simulink model "PassingDeadzone"  (R2023b)
settings: Solver=VariableStepAuto  StartTime=0.0  StopTime=20.0  FixedStep=.1  MaxStep=0.1  RelTol=1e-3
undefined symbols (not defined in the file or in its folder): Blue_Hub_LeftX, Blue_Hub_LeftY, Blue_Hub_RightX, Blue_Hub_RightY, Field_Length, Field_Length_Half, Field_Width, Rebuilt_Des_Gyro_Shoot_Offset
libraries: simulink_extras x3
settings Model: Creator=FIRSTMentor  LastModifiedBy=FIRSTMentor

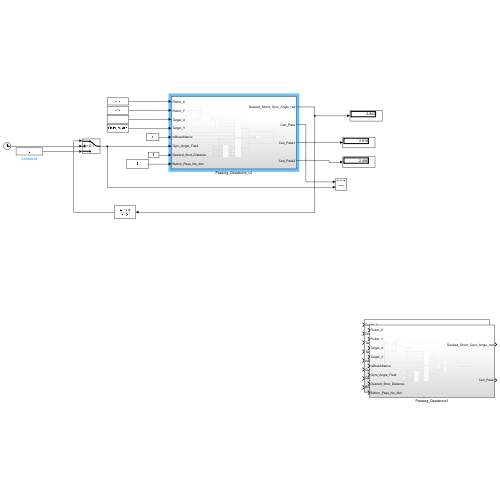
[thumbnail: Simulink's stored preview of the top-level diagram]
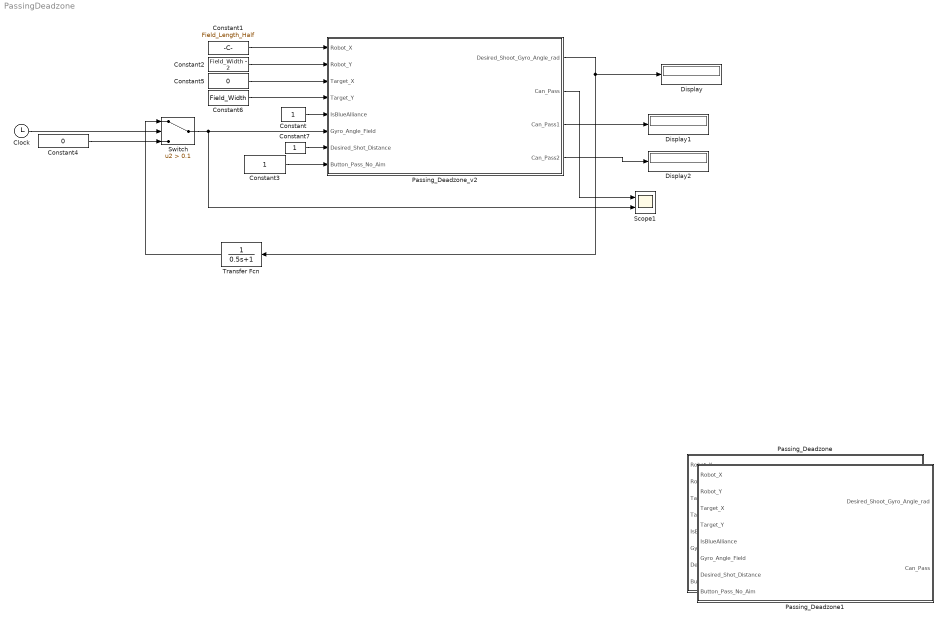
== system PassingDeadzone ==
  Clock : Clock
  Constant : Constant
  Constant1 : Constant  Value=Field_Length_Half
  Constant2 : Constant  Value=Field_Width - 2
  Constant3 : Constant
  Constant4 : Constant  Value=0
  Constant5 : Constant  Value=0
  Constant6 : Constant  Value=Field_Width
  Constant7 : Constant
  Display : Display
  Display1 : Display
  Display2 : Display
  Passing_Deadzone : Subsystem
  Passing_Deadzone1 : Subsystem
  Passing_Deadzone_v2 : Subsystem
  Scope1 : Scope  NumInputPorts=2
  Switch : Switch  Criteria=u2 > Threshold  Threshold=0.1  SaturateOnIntegerOverflow=off  InputSameDT=off
  Transfer Fcn : TransferFcn  Denominator=[0.5 1]
  wires:
  Constant/1 -> Passing_Deadzone_v2/5(IsBlueAlliance)
  Passing_Deadzone_v2/1(Desired_Shoot_Gyro_Angle_rad) -> Transfer Fcn/1, Display/1
  Passing_Deadzone_v2/2(Can_Pass) -> Scope1/1
  Constant3/1 -> Passing_Deadzone_v2/8(Button_Pass_No_Aim)
  Clock/1 -> Switch/2
  Constant4/1 -> Switch/3
  Transfer Fcn/1 -> Switch/1
  Switch/1 -> Scope1/2, Passing_Deadzone_v2/6(Gyro_Angle_Field)
  Constant1/1 -> Passing_Deadzone_v2/1(Robot_X)
  Constant2/1 -> Passing_Deadzone_v2/2(Robot_Y)
  Constant5/1 -> Passing_Deadzone_v2/3(Target_X)
  Constant6/1 -> Passing_Deadzone_v2/4(Target_Y)
  Constant7/1 -> Passing_Deadzone_v2/7(Desired_Shot_Distance)
  Passing_Deadzone_v2/3(Can_Pass1) -> Display1/1
  Passing_Deadzone_v2/4(Can_Pass2) -> Display2/1

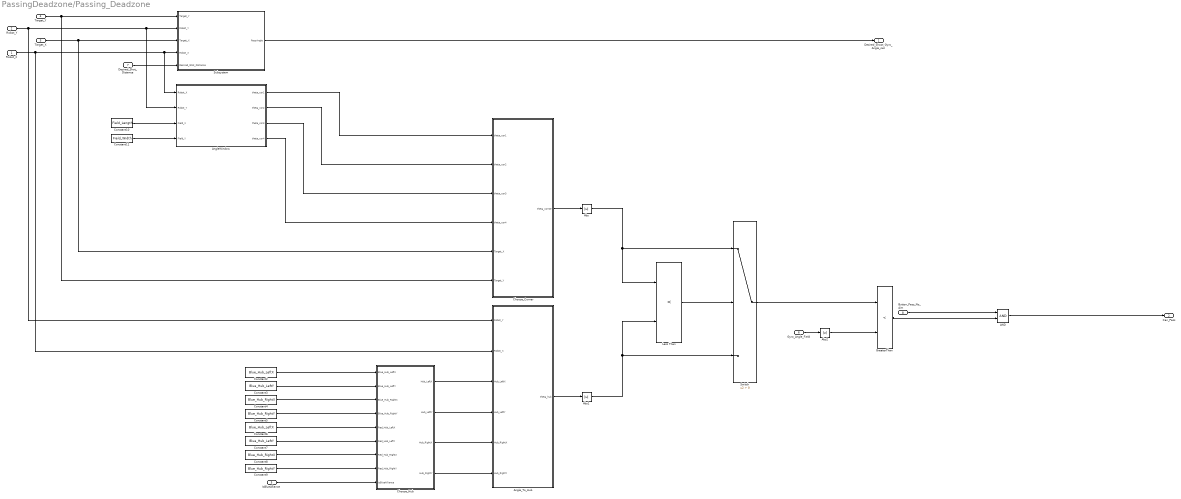
== system PassingDeadzone/Passing_Deadzone ==
  Robot_X : Inport
  Robot_Y : Inport  Port=2
  Target_X : Inport  Port=3
  Target_Y : Inport  Port=4
  IsBlueAlliance : Inport  Port=5
  Gyro_Angle_Field : Inport  Port=6
  Desired_Shot_Distance : Inport  Port=7
  Button_Pass_No_Aim : Inport  Port=8
  AND : Logic  AllPortsSameDT=off  OutDataTypeStr=boolean
  Abs : Abs  SaturateOnIntegerOverflow=off
  Abs1 : Abs  SaturateOnIntegerOverflow=off
  Abs2 : Abs  SaturateOnIntegerOverflow=off
  AngleWindow : Subsystem
  Angle_To_Hub : Subsystem
  Choose_Corner : Subsystem
  Choose_Hub : Subsystem
  Constant10 : Constant  Value=Field_Length
  Constant11 : Constant  Value=Field_Width
  Constant2 : Constant  Value=Blue_Hub_LeftX
  Constant3 : Constant  Value=Blue_Hub_LeftY
  Constant4 : Constant  Value=Blue_Hub_RightX
  Constant5 : Constant  Value=Blue_Hub_RightY
  Constant6 : Constant  Value=Blue_Hub_LeftX
  Constant7 : Constant  Value=Blue_Hub_LeftY
  Constant8 : Constant  Value=Blue_Hub_RightX
  Constant9 : Constant  Value=Blue_Hub_RightY
  GreaterThan : RelationalOperator  Operator=<  OutDataTypeStr=boolean  RndMeth=Simplest  InputSameDT=off
  Less Than : RelationalOperator  Operator=<  OutDataTypeStr=boolean  RndMeth=Simplest  InputSameDT=off
  Subsystem : Subsystem
  Switch : Switch  Criteria=u2 > Threshold  SaturateOnIntegerOverflow=off  InputSameDT=off
  Desired_Shoot_Gyro_Angle_rad : Outport
  Can_Pass : Outport  Port=2
  wires:
  Target_Y/1 -> Choose_Corner/6(Target_Y), Subsystem/1(Target_Y)
  Robot_Y/1 -> Angle_To_Hub/1(Robot_Y), AngleWindow/2(Robot_Y), Subsystem/2(Robot_Y)
  Target_X/1 -> Choose_Corner/5(Target_X), Subsystem/3(Target_X)
  Robot_X/1 -> AngleWindow/1(Robot_X), Subsystem/4(Robot_X), Angle_To_Hub/2(Robot_X)
  Constant10/1 -> AngleWindow/3(Field_X)
  AngleWindow/1(theta_cor1) -> Choose_Corner/1(theta_cor1)
  AngleWindow/2(theta_cor2) -> Choose_Corner/2(theta_cor2)
  AngleWindow/3(theta_cor3) -> Choose_Corner/3(theta_cor3)
  AngleWindow/4(theta_cor4) -> Choose_Corner/4(theta_cor4)
  Constant2/1 -> Choose_Hub/1(Blue_Hub_LeftX)
  Constant4/1 -> Choose_Hub/3(Blue_Hub_RightX)
  Constant5/1 -> Choose_Hub/4(Blue_Hub_RightY)
  Constant6/1 -> Choose_Hub/5(Red_Hub_LeftX)
  Constant7/1 -> Choose_Hub/6(Red_Hub_LeftY)
  Constant8/1 -> Choose_Hub/7(Red_Hub_RightX)
  Constant9/1 -> Choose_Hub/8(Red_Hub_RightY)
  IsBlueAlliance/1 -> Choose_Hub/9(IsBlueAlliance)
  Choose_Hub/1(Hub_LeftX) -> Angle_To_Hub/3(Hub_LeftX)
  Choose_Hub/2(Hub_LeftY) -> Angle_To_Hub/4(Hub_LeftY)
  Choose_Hub/3(Hub_RightX) -> Angle_To_Hub/5(Hub_RightX)
  Choose_Hub/4(Hub_RightY) -> Angle_To_Hub/6(Hub_RightY)
  Choose_Corner/1(theta_corner) -> Abs/1
  Angle_To_Hub/1(theta_hub) -> Abs1/1
  Abs/1 -> Switch/1, Less Than/1
  Abs1/1 -> Switch/3, Less Than/2
  Less Than/1 -> Switch/2
  Switch/1 -> GreaterThan/1
  Gyro_Angle_Field/1 -> Abs2/1
  Subsystem/1(PassAngle) -> Desired_Shoot_Gyro_Angle_rad/1
  Abs2/1 -> GreaterThan/2
  Constant3/1 -> Choose_Hub/2(Blue_Hub_LeftY)
  Constant11/1 -> AngleWindow/4(Field_Y)
  Desired_Shot_Distance/1 -> Subsystem/5(Desired_Shot_Distance)
  AND/1 -> Can_Pass/1
  Button_Pass_No_Aim/1 -> AND/1
  GreaterThan/1 -> AND/2

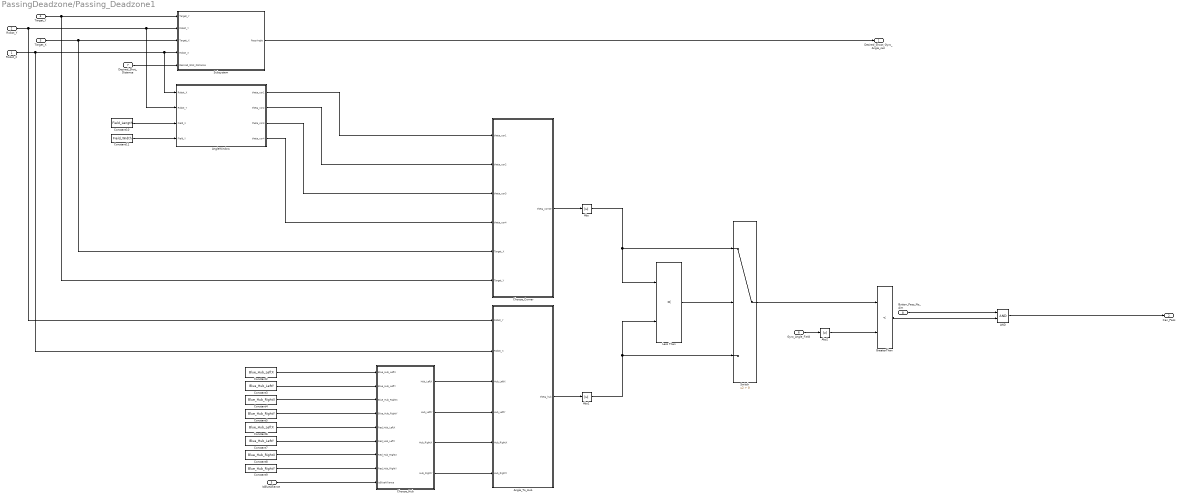
== system PassingDeadzone/Passing_Deadzone1 ==
  Robot_X : Inport
  Robot_Y : Inport  Port=2
  Target_X : Inport  Port=3
  Target_Y : Inport  Port=4
  IsBlueAlliance : Inport  Port=5
  Gyro_Angle_Field : Inport  Port=6
  Desired_Shot_Distance : Inport  Port=7
  Button_Pass_No_Aim : Inport  Port=8
  AND : Logic  AllPortsSameDT=off  OutDataTypeStr=boolean
  Abs : Abs  SaturateOnIntegerOverflow=off
  Abs1 : Abs  SaturateOnIntegerOverflow=off
  Abs2 : Abs  SaturateOnIntegerOverflow=off
  AngleWindow : Subsystem
  Angle_To_Hub : Subsystem
  Choose_Corner : Subsystem
  Choose_Hub : Subsystem
  Constant10 : Constant  Value=Field_Length
  Constant11 : Constant  Value=Field_Width
  Constant2 : Constant  Value=Blue_Hub_LeftX
  Constant3 : Constant  Value=Blue_Hub_LeftY
  Constant4 : Constant  Value=Blue_Hub_RightX
  Constant5 : Constant  Value=Blue_Hub_RightY
  Constant6 : Constant  Value=Blue_Hub_LeftX
  Constant7 : Constant  Value=Blue_Hub_LeftY
  Constant8 : Constant  Value=Blue_Hub_RightX
  Constant9 : Constant  Value=Blue_Hub_RightY
  GreaterThan : RelationalOperator  Operator=<  OutDataTypeStr=boolean  RndMeth=Simplest  InputSameDT=off
  Less Than : RelationalOperator  Operator=<  OutDataTypeStr=boolean  RndMeth=Simplest  InputSameDT=off
  Subsystem : Subsystem
  Switch : Switch  Criteria=u2 > Threshold  SaturateOnIntegerOverflow=off  InputSameDT=off
  Desired_Shoot_Gyro_Angle_rad : Outport
  Can_Pass : Outport  Port=2
  wires:
  Target_Y/1 -> Choose_Corner/6(Target_Y), Subsystem/1(Target_Y)
  Robot_Y/1 -> Angle_To_Hub/1(Robot_Y), AngleWindow/2(Robot_Y), Subsystem/2(Robot_Y)
  Target_X/1 -> Choose_Corner/5(Target_X), Subsystem/3(Target_X)
  Robot_X/1 -> AngleWindow/1(Robot_X), Subsystem/4(Robot_X), Angle_To_Hub/2(Robot_X)
  Constant10/1 -> AngleWindow/3(Field_X)
  AngleWindow/1(theta_cor1) -> Choose_Corner/1(theta_cor1)
  AngleWindow/2(theta_cor2) -> Choose_Corner/2(theta_cor2)
  AngleWindow/3(theta_cor3) -> Choose_Corner/3(theta_cor3)
  AngleWindow/4(theta_cor4) -> Choose_Corner/4(theta_cor4)
  Constant2/1 -> Choose_Hub/1(Blue_Hub_LeftX)
  Constant4/1 -> Choose_Hub/3(Blue_Hub_RightX)
  Constant5/1 -> Choose_Hub/4(Blue_Hub_RightY)
  Constant6/1 -> Choose_Hub/5(Red_Hub_LeftX)
  Constant7/1 -> Choose_Hub/6(Red_Hub_LeftY)
  Constant8/1 -> Choose_Hub/7(Red_Hub_RightX)
  Constant9/1 -> Choose_Hub/8(Red_Hub_RightY)
  IsBlueAlliance/1 -> Choose_Hub/9(IsBlueAlliance)
  Choose_Hub/1(Hub_LeftX) -> Angle_To_Hub/3(Hub_LeftX)
  Choose_Hub/2(Hub_LeftY) -> Angle_To_Hub/4(Hub_LeftY)
  Choose_Hub/3(Hub_RightX) -> Angle_To_Hub/5(Hub_RightX)
  Choose_Hub/4(Hub_RightY) -> Angle_To_Hub/6(Hub_RightY)
  Choose_Corner/1(theta_corner) -> Abs/1
  Angle_To_Hub/1(theta_hub) -> Abs1/1
  Abs/1 -> Switch/1, Less Than/1
  Abs1/1 -> Switch/3, Less Than/2
  Less Than/1 -> Switch/2
  Switch/1 -> GreaterThan/1
  Gyro_Angle_Field/1 -> Abs2/1
  Subsystem/1(PassAngle) -> Desired_Shoot_Gyro_Angle_rad/1
  Abs2/1 -> GreaterThan/2
  Constant3/1 -> Choose_Hub/2(Blue_Hub_LeftY)
  Constant11/1 -> AngleWindow/4(Field_Y)
  Desired_Shot_Distance/1 -> Subsystem/5(Desired_Shot_Distance)
  AND/1 -> Can_Pass/1
  Button_Pass_No_Aim/1 -> AND/1
  GreaterThan/1 -> AND/2

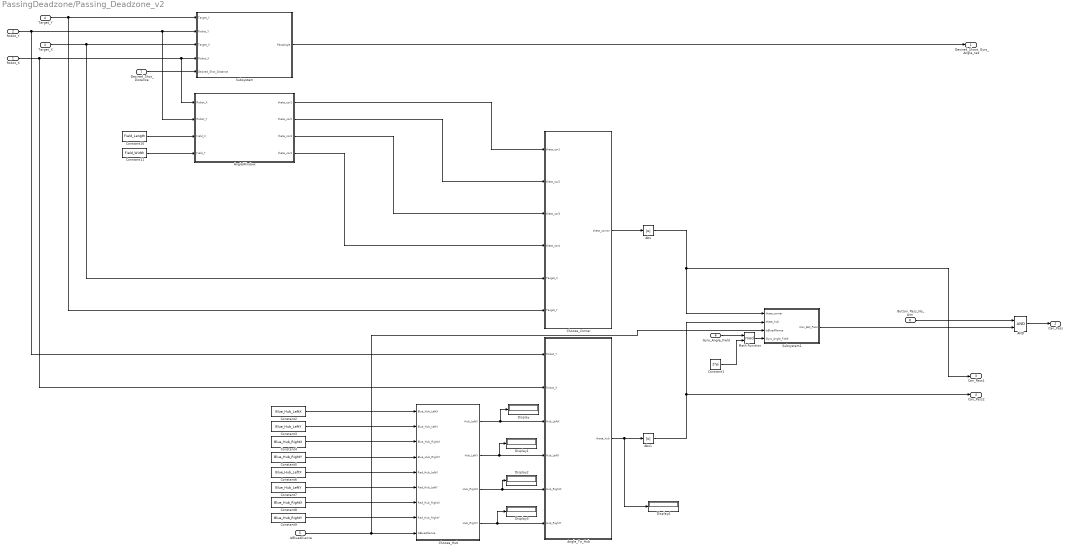
== system PassingDeadzone/Passing_Deadzone_v2 ==
  Robot_X : Inport
  Robot_Y : Inport  Port=2
  Target_X : Inport  Port=3
  Target_Y : Inport  Port=4
  IsBlueAlliance : Inport  Port=5
  Gyro_Angle_Field : Inport  Port=6
  Desired_Shot_Distance : Inport  Port=7
  Button_Pass_No_Aim : Inport  Port=8
  AND : Logic  AllPortsSameDT=off  OutDataTypeStr=boolean
  Abs : Abs  SaturateOnIntegerOverflow=off
  Abs1 : Abs  SaturateOnIntegerOverflow=off
  AngleWindow : Subsystem
  Angle_To_Hub : Subsystem
  Choose_Corner : Subsystem
  Choose_Hub : Subsystem
  Constant1 : Constant  Value=2*pi
  Constant10 : Constant  Value=Field_Length
  Constant11 : Constant  Value=Field_Width
  Constant2 : Constant  Value=Blue_Hub_LeftX
  Constant3 : Constant  Value=Blue_Hub_LeftY
  Constant4 : Constant  Value=Blue_Hub_RightX
  Constant5 : Constant  Value=Blue_Hub_RightY
  Constant6 : Constant  Value=Blue_Hub_LeftX
  Constant7 : Constant  Value=Blue_Hub_LeftY
  Constant8 : Constant  Value=Blue_Hub_RightX
  Constant9 : Constant  Value=Blue_Hub_RightY
  Display{,1..4} (5 alike) : Display
  Math Function : Math  Operator=mod
  Subsystem : Subsystem
  Subsystem1 : Subsystem
  Desired_Shoot_Gyro_Angle_rad : Outport
  Can_Pass : Outport  Port=2
  Can_Pass1 : Outport  Port=3
  Can_Pass2 : Outport  Port=4
  wires:
  Target_Y/1 -> Choose_Corner/6(Target_Y), Subsystem/1(Target_Y)
  Robot_Y/1 -> Angle_To_Hub/1(Robot_Y), AngleWindow/2(Robot_Y), Subsystem/2(Robot_Y)
  Target_X/1 -> Choose_Corner/5(Target_X), Subsystem/3(Target_X)
  Robot_X/1 -> AngleWindow/1(Robot_X), Subsystem/4(Robot_X), Angle_To_Hub/2(Robot_X)
  Constant10/1 -> AngleWindow/3(Field_X)
  AngleWindow/1(theta_cor1) -> Choose_Corner/1(theta_cor1)
  AngleWindow/2(theta_cor2) -> Choose_Corner/2(theta_cor2)
  AngleWindow/3(theta_cor3) -> Choose_Corner/3(theta_cor3)
  AngleWindow/4(theta_cor4) -> Choose_Corner/4(theta_cor4)
  Constant2/1 -> Choose_Hub/1(Blue_Hub_LeftX)
  Constant4/1 -> Choose_Hub/3(Blue_Hub_RightX)
  Constant5/1 -> Choose_Hub/4(Blue_Hub_RightY)
  Constant6/1 -> Choose_Hub/5(Red_Hub_LeftX)
  Constant7/1 -> Choose_Hub/6(Red_Hub_LeftY)
  Constant8/1 -> Choose_Hub/7(Red_Hub_RightX)
  Constant9/1 -> Choose_Hub/8(Red_Hub_RightY)
  IsBlueAlliance/1 -> Subsystem1/3(IsBlueAlliance), Choose_Hub/9(IsBlueAlliance)
  Choose_Hub/1(Hub_LeftX) -> Display/1, Angle_To_Hub/3(Hub_LeftX)
  Choose_Hub/2(Hub_LeftY) -> Display1/1, Angle_To_Hub/4(Hub_LeftY)
  Choose_Hub/3(Hub_RightX) -> Display2/1, Angle_To_Hub/5(Hub_RightX)
  Choose_Hub/4(Hub_RightY) -> Display3/1, Angle_To_Hub/6(Hub_RightY)
  Choose_Corner/1(theta_corner) -> Abs/1
  Angle_To_Hub/1(theta_hub) -> Display4/1, Abs1/1
  Subsystem/1(PassAngle) -> Desired_Shoot_Gyro_Angle_rad/1
  Constant3/1 -> Choose_Hub/2(Blue_Hub_LeftY)
  Constant11/1 -> AngleWindow/4(Field_Y)
  Desired_Shot_Distance/1 -> Subsystem/5(Desired_Shot_Distance)
  AND/1 -> Can_Pass/1
  Abs/1 -> Can_Pass1/1, Subsystem1/1(theta_corner)
  Abs1/1 -> Can_Pass2/1, Subsystem1/2(theta_hub)
  Subsystem1/1(Can_Bot_Pass) -> AND/2
  Constant1/1 -> Math Function/2
  Gyro_Angle_Field/1 -> Math Function/1
  Math Function/1 -> Subsystem1/4(Gyro_Angle_Field)
  Button_Pass_No_Aim/1 -> AND/1

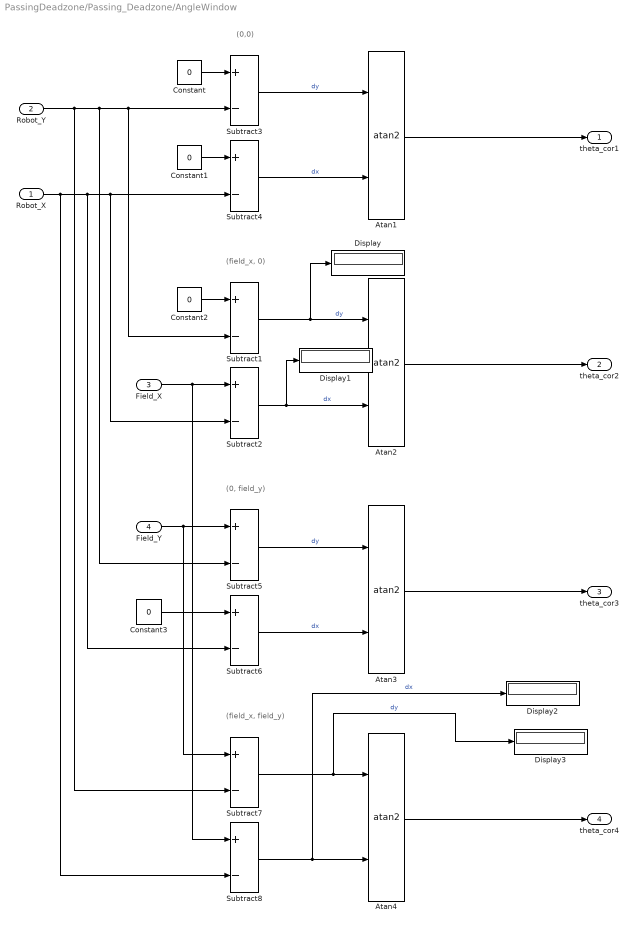
== system PassingDeadzone/Passing_Deadzone/AngleWindow ==
  note: (0,0)
  note: (field_x, 0)
  note: (0, field_y)
  note: (field_x, field_y)
  Robot_X : Inport
  Robot_Y : Inport  Port=2
  Field_X : Inport  Port=3
  Field_Y : Inport  Port=4
  Atan{1..4} (4 alike) : Trigonometry  Operator=atan2
  Constant{,1..3} (4 alike) : Constant  Value=0
  Display{,1..3} (4 alike) : Display
  Subtract{1..8} (8 alike) : Sum  Inputs=+-
  theta_cor1 : Outport
  theta_cor2 : Outport  Port=2
  theta_cor3 : Outport  Port=3
  theta_cor4 : Outport  Port=4
  wires:
  Subtract3/1 -> Atan1/1  "dy"
  Subtract4/1 -> Atan1/2  "dx"
  Atan1/1 -> theta_cor1/1
  Subtract1/1 -> Display/1, Atan2/1  "dy"
  Subtract2/1 -> Display1/1, Atan2/2  "dx"
  Atan2/1 -> theta_cor2/1
  Subtract5/1 -> Atan3/1  "dy"
  Subtract6/1 -> Atan3/2  "dx"
  Atan3/1 -> theta_cor3/1
  Subtract7/1 -> Display3/1, Atan4/1  "dy"
  Subtract8/1 -> Display2/1, Atan4/2  "dx"
  Atan4/1 -> theta_cor4/1
  Constant/1 -> Subtract3/1
  Constant1/1 -> Subtract4/1
  Robot_Y/1 -> Subtract7/2, Subtract1/2, Subtract3/2, Subtract5/2
  Robot_X/1 -> Subtract8/2, Subtract6/2, Subtract2/2, Subtract4/2
  Field_X/1 -> Subtract8/1, Subtract2/1
  Constant2/1 -> Subtract1/1
  Field_Y/1 -> Subtract7/1, Subtract5/1
  Constant3/1 -> Subtract6/1

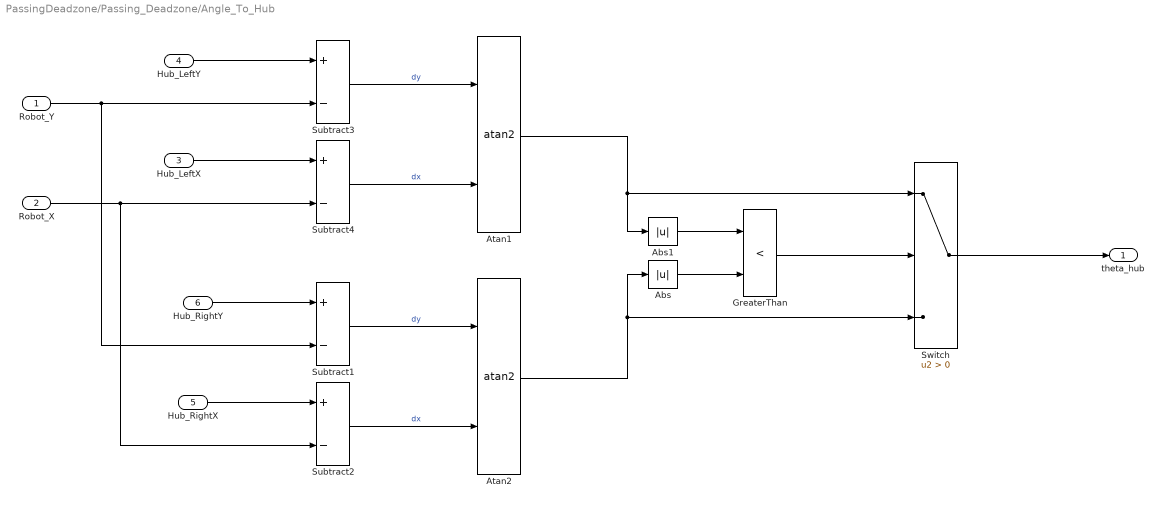
== system PassingDeadzone/Passing_Deadzone/Angle_To_Hub ==
  Robot_Y : Inport
  Robot_X : Inport  Port=2
  Hub_LeftX : Inport  Port=3
  Hub_LeftY : Inport  Port=4
  Hub_RightX : Inport  Port=5
  Hub_RightY : Inport  Port=6
  Abs : Abs  SaturateOnIntegerOverflow=off
  Abs1 : Abs  SaturateOnIntegerOverflow=off
  Atan1 : Trigonometry  Operator=atan2
  Atan2 : Trigonometry  Operator=atan2
  GreaterThan : RelationalOperator  Operator=<  OutDataTypeStr=boolean  RndMeth=Simplest  InputSameDT=off
  Subtract{1..4} (4 alike) : Sum  Inputs=+-
  Switch : Switch  Criteria=u2 > Threshold  SaturateOnIntegerOverflow=off  InputSameDT=off
  theta_hub : Outport
  wires:
  Subtract4/1 -> Atan1/2  "dx"
  Subtract3/1 -> Atan1/1  "dy"
  Robot_Y/1 -> Subtract3/2, Subtract1/2
  Robot_X/1 -> Subtract4/2, Subtract2/2
  Hub_LeftY/1 -> Subtract3/1
  Hub_LeftX/1 -> Subtract4/1
  Subtract1/1 -> Atan2/1  "dy"
  Subtract2/1 -> Atan2/2  "dx"
  Hub_RightX/1 -> Subtract2/1
  Hub_RightY/1 -> Subtract1/1
  Atan2/1 -> Switch/3, Abs/1
  Atan1/1 -> Switch/1, Abs1/1
  GreaterThan/1 -> Switch/2
  Switch/1 -> theta_hub/1
  Abs1/1 -> GreaterThan/1
  Abs/1 -> GreaterThan/2

== system PassingDeadzone/Passing_Deadzone/Choose_Corner ==
  theta_cor1 : Inport
  theta_cor2 : Inport  Port=2
  theta_cor3 : Inport  Port=3
  theta_cor4 : Inport  Port=4
  Target_X : Inport  Port=5
  Target_Y : Inport  Port=6
  If : If  IfExpression=u1 > Field_Hub_Y
  If Action Subsystem : Subsystem  TreatAsAtomicUnit=on
  If Action Subsystem1 : Subsystem  TreatAsAtomicUnit=on
  Merge : Merge
  theta_corner : Outport
  wires:
  If/1 -> If Action Subsystem/Action
  Target_Y/1 -> If/1
  If/2 -> If Action Subsystem1/Action
  theta_cor1/1 -> If Action Subsystem1/1(theta_cor1)
  If Action Subsystem/1(theta_corner) -> Merge/1
  If Action Subsystem1/1(theta_corner) -> Merge/2
  Merge/1 -> theta_corner/1
  Target_X/1 -> If Action Subsystem1/3(Target_X), If Action Subsystem/3(Target_X)
  theta_cor2/1 -> If Action Subsystem1/2(theta_cor2)
  theta_cor3/1 -> If Action Subsystem/1(theta_cor3)
  theta_cor4/1 -> If Action Subsystem/2(theta_cor4)

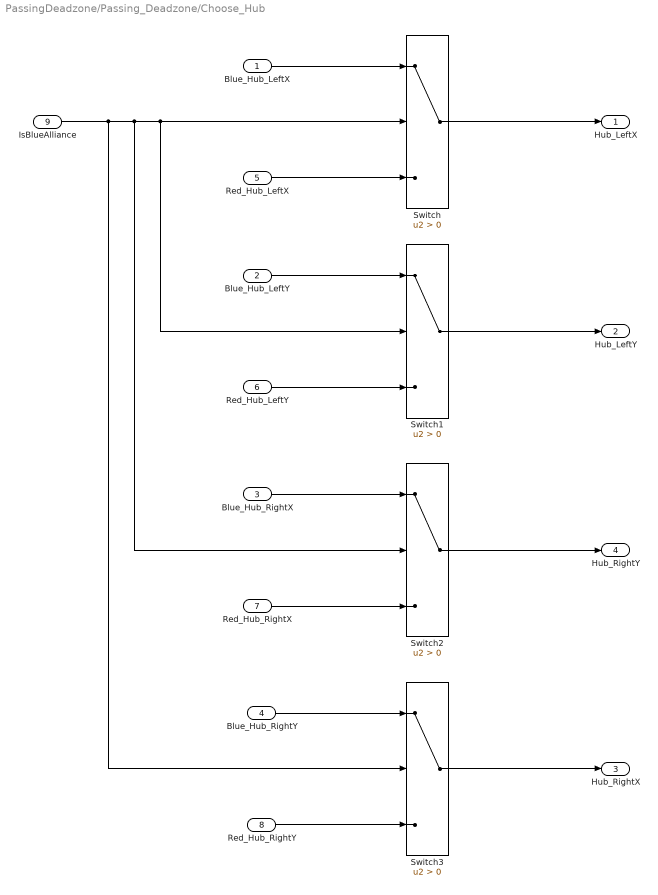
== system PassingDeadzone/Passing_Deadzone/Choose_Hub ==
  Blue_Hub_LeftX : Inport
  Blue_Hub_LeftY : Inport  Port=2
  Blue_Hub_RightX : Inport  Port=3
  Blue_Hub_RightY : Inport  Port=4
  Red_Hub_LeftX : Inport  Port=5
  Red_Hub_LeftY : Inport  Port=6
  Red_Hub_RightX : Inport  Port=7
  Red_Hub_RightY : Inport  Port=8
  IsBlueAlliance : Inport  Port=9
  Switch{,1..3} (4 alike) : Switch  Criteria=u2 > Threshold  SaturateOnIntegerOverflow=off  InputSameDT=off
  Hub_LeftX : Outport
  Hub_LeftY : Outport  Port=2
  Hub_RightX : Outport  Port=3
  Hub_RightY : Outport  Port=4
  wires:
  IsBlueAlliance/1 -> Switch/2, Switch1/2, Switch2/2, Switch3/2
  Switch/1 -> Hub_LeftX/1
  Switch1/1 -> Hub_LeftY/1
  Switch2/1 -> Hub_RightY/1
  Switch3/1 -> Hub_RightX/1
  Blue_Hub_LeftX/1 -> Switch/1
  Red_Hub_LeftY/1 -> Switch1/3
  Blue_Hub_LeftY/1 -> Switch1/1
  Blue_Hub_RightX/1 -> Switch2/1
  Red_Hub_RightX/1 -> Switch2/3
  Red_Hub_RightY/1 -> Switch3/3
  Blue_Hub_RightY/1 -> Switch3/1
  Red_Hub_LeftX/1 -> Switch/3

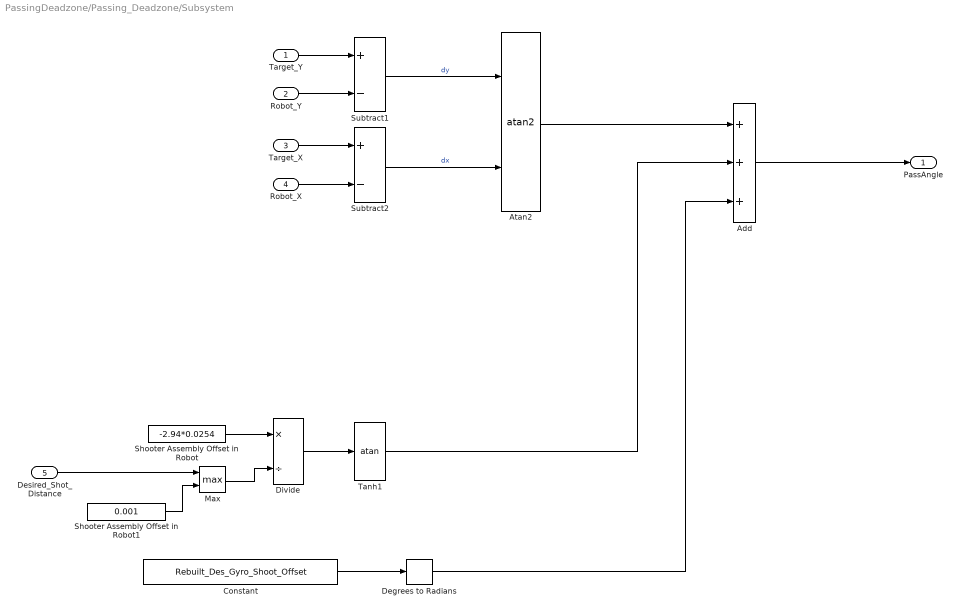
== system PassingDeadzone/Passing_Deadzone/Subsystem ==
  Target_Y : Inport
  Robot_Y : Inport  Port=2
  Target_X : Inport  Port=3
  Robot_X : Inport  Port=4
  Desired_Shot_Distance : Inport  Port=5
  Add : Sum  Inputs=+++
  Atan2 : Trigonometry  Operator=atan2
  Constant : Constant  Value=Rebuilt_Des_Gyro_Shoot_Offset
  Degrees to Radians : simulink_extras/Transformations/Degrees to Radians
  Divide : Product  Inputs=*/
  Max : MinMax  Function=max  Inputs=2
  Shooter Assembly Offset in Robot : Constant  Value=-2.94*0.0254
  Shooter Assembly Offset in Robot1 : Constant  Value=0.001
  Subtract1 : Sum  Inputs=+-
  Subtract2 : Sum  Inputs=+-
  Tanh1 : Trigonometry  Operator=atan
  PassAngle : Outport
  wires:
  Target_X/1 -> Subtract2/1
  Subtract2/1 -> Atan2/2  "dx"
  Subtract1/1 -> Atan2/1  "dy"
  Target_Y/1 -> Subtract1/1
  Robot_X/1 -> Subtract2/2
  Robot_Y/1 -> Subtract1/2
  Max/1 -> Divide/2
  Shooter Assembly Offset in Robot/1 -> Divide/1
  Shooter Assembly Offset in Robot1/1 -> Max/2
  Divide/1 -> Tanh1/1
  Desired_Shot_Distance/1 -> Max/1
  Tanh1/1 -> Add/2
  Constant/1 -> Degrees to Radians/1
  Add/1 -> PassAngle/1
  Atan2/1 -> Add/1
  Degrees to Radians/1 -> Add/3

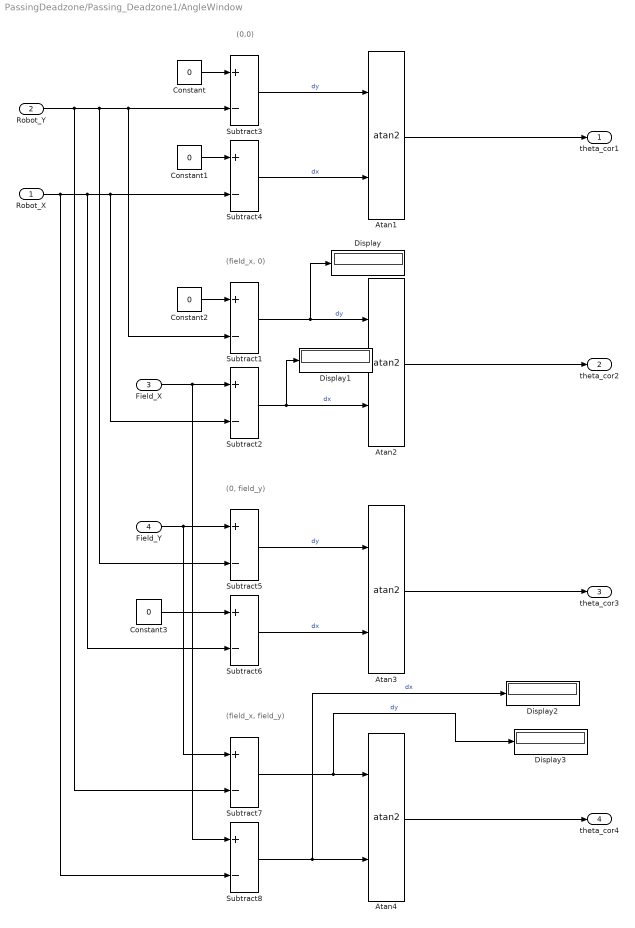
== system PassingDeadzone/Passing_Deadzone1/AngleWindow ==
  note: (0,0)
  note: (field_x, 0)
  note: (0, field_y)
  note: (field_x, field_y)
  Robot_X : Inport
  Robot_Y : Inport  Port=2
  Field_X : Inport  Port=3
  Field_Y : Inport  Port=4
  Atan{1..4} (4 alike) : Trigonometry  Operator=atan2
  Constant{,1..3} (4 alike) : Constant  Value=0
  Display{,1..3} (4 alike) : Display
  Subtract{1..8} (8 alike) : Sum  Inputs=+-
  theta_cor1 : Outport
  theta_cor2 : Outport  Port=2
  theta_cor3 : Outport  Port=3
  theta_cor4 : Outport  Port=4
  wires:
  Subtract3/1 -> Atan1/1  "dy"
  Subtract4/1 -> Atan1/2  "dx"
  Atan1/1 -> theta_cor1/1
  Subtract1/1 -> Display/1, Atan2/1  "dy"
  Subtract2/1 -> Display1/1, Atan2/2  "dx"
  Atan2/1 -> theta_cor2/1
  Subtract5/1 -> Atan3/1  "dy"
  Subtract6/1 -> Atan3/2  "dx"
  Atan3/1 -> theta_cor3/1
  Subtract7/1 -> Display3/1, Atan4/1  "dy"
  Subtract8/1 -> Display2/1, Atan4/2  "dx"
  Atan4/1 -> theta_cor4/1
  Constant/1 -> Subtract3/1
  Constant1/1 -> Subtract4/1
  Robot_Y/1 -> Subtract7/2, Subtract1/2, Subtract3/2, Subtract5/2
  Robot_X/1 -> Subtract8/2, Subtract6/2, Subtract2/2, Subtract4/2
  Field_X/1 -> Subtract8/1, Subtract2/1
  Constant2/1 -> Subtract1/1
  Field_Y/1 -> Subtract7/1, Subtract5/1
  Constant3/1 -> Subtract6/1

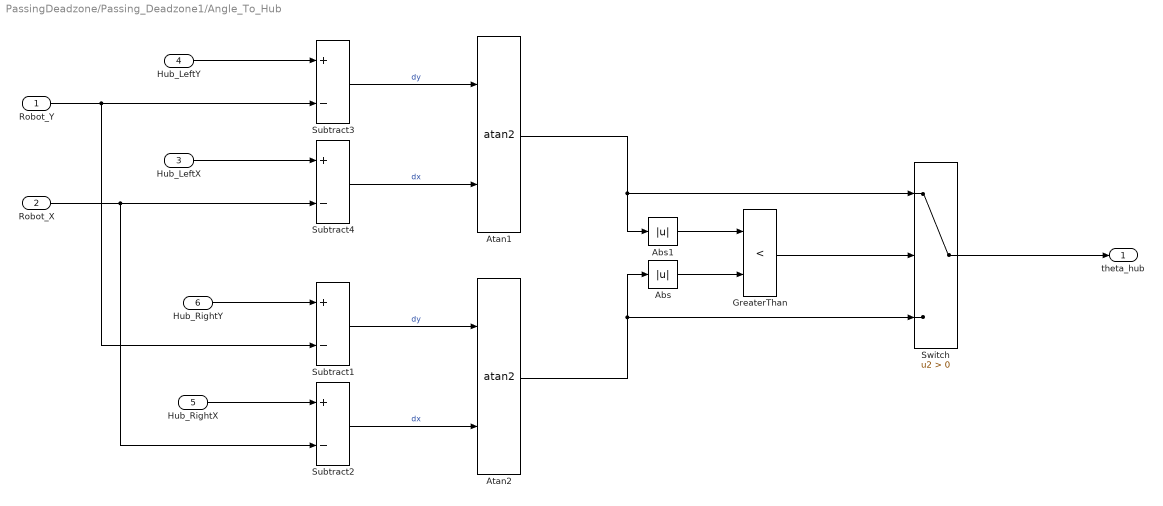
== system PassingDeadzone/Passing_Deadzone1/Angle_To_Hub ==
  Robot_Y : Inport
  Robot_X : Inport  Port=2
  Hub_LeftX : Inport  Port=3
  Hub_LeftY : Inport  Port=4
  Hub_RightX : Inport  Port=5
  Hub_RightY : Inport  Port=6
  Abs : Abs  SaturateOnIntegerOverflow=off
  Abs1 : Abs  SaturateOnIntegerOverflow=off
  Atan1 : Trigonometry  Operator=atan2
  Atan2 : Trigonometry  Operator=atan2
  GreaterThan : RelationalOperator  Operator=<  OutDataTypeStr=boolean  RndMeth=Simplest  InputSameDT=off
  Subtract{1..4} (4 alike) : Sum  Inputs=+-
  Switch : Switch  Criteria=u2 > Threshold  SaturateOnIntegerOverflow=off  InputSameDT=off
  theta_hub : Outport
  wires:
  Subtract4/1 -> Atan1/2  "dx"
  Subtract3/1 -> Atan1/1  "dy"
  Robot_Y/1 -> Subtract3/2, Subtract1/2
  Robot_X/1 -> Subtract4/2, Subtract2/2
  Hub_LeftY/1 -> Subtract3/1
  Hub_LeftX/1 -> Subtract4/1
  Subtract1/1 -> Atan2/1  "dy"
  Subtract2/1 -> Atan2/2  "dx"
  Hub_RightX/1 -> Subtract2/1
  Hub_RightY/1 -> Subtract1/1
  Atan2/1 -> Switch/3, Abs/1
  Atan1/1 -> Switch/1, Abs1/1
  GreaterThan/1 -> Switch/2
  Switch/1 -> theta_hub/1
  Abs1/1 -> GreaterThan/1
  Abs/1 -> GreaterThan/2

== system PassingDeadzone/Passing_Deadzone1/Choose_Corner ==
  theta_cor1 : Inport
  theta_cor2 : Inport  Port=2
  theta_cor3 : Inport  Port=3
  theta_cor4 : Inport  Port=4
  Target_X : Inport  Port=5
  Target_Y : Inport  Port=6
  If : If  IfExpression=u1 > Field_Hub_Y
  If Action Subsystem : Subsystem  TreatAsAtomicUnit=on
  If Action Subsystem1 : Subsystem  TreatAsAtomicUnit=on
  Merge : Merge
  theta_corner : Outport
  wires:
  If/1 -> If Action Subsystem/Action
  Target_Y/1 -> If/1
  If/2 -> If Action Subsystem1/Action
  theta_cor1/1 -> If Action Subsystem1/1(theta_cor1)
  If Action Subsystem/1(theta_corner) -> Merge/1
  If Action Subsystem1/1(theta_corner) -> Merge/2
  Merge/1 -> theta_corner/1
  Target_X/1 -> If Action Subsystem1/3(Target_X), If Action Subsystem/3(Target_X)
  theta_cor2/1 -> If Action Subsystem1/2(theta_cor2)
  theta_cor3/1 -> If Action Subsystem/1(theta_cor3)
  theta_cor4/1 -> If Action Subsystem/2(theta_cor4)

== system PassingDeadzone/Passing_Deadzone1/Choose_Hub ==
  Blue_Hub_LeftX : Inport
  Blue_Hub_LeftY : Inport  Port=2
  Blue_Hub_RightX : Inport  Port=3
  Blue_Hub_RightY : Inport  Port=4
  Red_Hub_LeftX : Inport  Port=5
  Red_Hub_LeftY : Inport  Port=6
  Red_Hub_RightX : Inport  Port=7
  Red_Hub_RightY : Inport  Port=8
  IsBlueAlliance : Inport  Port=9
  Switch{,1..3} (4 alike) : Switch  Criteria=u2 > Threshold  SaturateOnIntegerOverflow=off  InputSameDT=off
  Hub_LeftX : Outport
  Hub_LeftY : Outport  Port=2
  Hub_RightX : Outport  Port=3
  Hub_RightY : Outport  Port=4
  wires:
  IsBlueAlliance/1 -> Switch/2, Switch1/2, Switch2/2, Switch3/2
  Switch/1 -> Hub_LeftX/1
  Switch1/1 -> Hub_LeftY/1
  Switch2/1 -> Hub_RightY/1
  Switch3/1 -> Hub_RightX/1
  Blue_Hub_LeftX/1 -> Switch/1
  Red_Hub_LeftY/1 -> Switch1/3
  Blue_Hub_LeftY/1 -> Switch1/1
  Blue_Hub_RightX/1 -> Switch2/1
  Red_Hub_RightX/1 -> Switch2/3
  Red_Hub_RightY/1 -> Switch3/3
  Blue_Hub_RightY/1 -> Switch3/1
  Red_Hub_LeftX/1 -> Switch/3

== system PassingDeadzone/Passing_Deadzone1/Subsystem ==
  Target_Y : Inport
  Robot_Y : Inport  Port=2
  Target_X : Inport  Port=3
  Robot_X : Inport  Port=4
  Desired_Shot_Distance : Inport  Port=5
  Add : Sum  Inputs=+++
  Atan2 : Trigonometry  Operator=atan2
  Constant : Constant  Value=Rebuilt_Des_Gyro_Shoot_Offset
  Degrees to Radians : simulink_extras/Transformations/Degrees to Radians
  Divide : Product  Inputs=*/
  Max : MinMax  Function=max  Inputs=2
  Shooter Assembly Offset in Robot : Constant  Value=-2.94*0.0254
  Shooter Assembly Offset in Robot1 : Constant  Value=0.001
  Subtract1 : Sum  Inputs=+-
  Subtract2 : Sum  Inputs=+-
  Tanh1 : Trigonometry  Operator=atan
  PassAngle : Outport
  wires:
  Target_X/1 -> Subtract2/1
  Subtract2/1 -> Atan2/2  "dx"
  Subtract1/1 -> Atan2/1  "dy"
  Target_Y/1 -> Subtract1/1
  Robot_X/1 -> Subtract2/2
  Robot_Y/1 -> Subtract1/2
  Max/1 -> Divide/2
  Shooter Assembly Offset in Robot/1 -> Divide/1
  Shooter Assembly Offset in Robot1/1 -> Max/2
  Divide/1 -> Tanh1/1
  Desired_Shot_Distance/1 -> Max/1
  Tanh1/1 -> Add/2
  Constant/1 -> Degrees to Radians/1
  Add/1 -> PassAngle/1
  Atan2/1 -> Add/1
  Degrees to Radians/1 -> Add/3

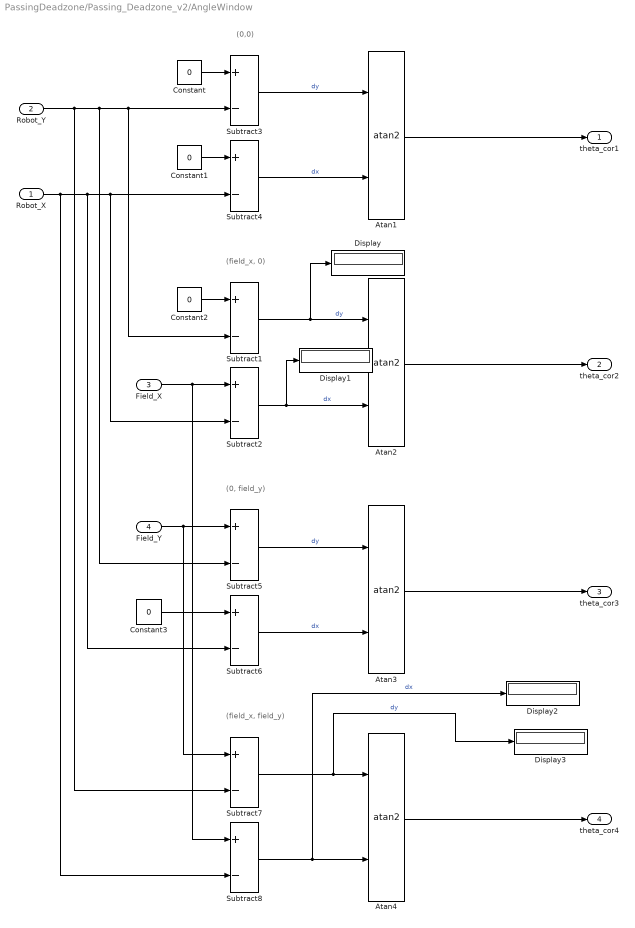
== system PassingDeadzone/Passing_Deadzone_v2/AngleWindow ==
  note: (0,0)
  note: (field_x, 0)
  note: (0, field_y)
  note: (field_x, field_y)
  Robot_X : Inport
  Robot_Y : Inport  Port=2
  Field_X : Inport  Port=3
  Field_Y : Inport  Port=4
  Atan{1..4} (4 alike) : Trigonometry  Operator=atan2
  Constant{,1..3} (4 alike) : Constant  Value=0
  Display{,1..3} (4 alike) : Display
  Subtract{1..8} (8 alike) : Sum  Inputs=+-
  theta_cor1 : Outport
  theta_cor2 : Outport  Port=2
  theta_cor3 : Outport  Port=3
  theta_cor4 : Outport  Port=4
  wires:
  Subtract3/1 -> Atan1/1  "dy"
  Subtract4/1 -> Atan1/2  "dx"
  Atan1/1 -> theta_cor1/1
  Subtract1/1 -> Display/1, Atan2/1  "dy"
  Subtract2/1 -> Display1/1, Atan2/2  "dx"
  Atan2/1 -> theta_cor2/1
  Subtract5/1 -> Atan3/1  "dy"
  Subtract6/1 -> Atan3/2  "dx"
  Atan3/1 -> theta_cor3/1
  Subtract7/1 -> Display3/1, Atan4/1  "dy"
  Subtract8/1 -> Display2/1, Atan4/2  "dx"
  Atan4/1 -> theta_cor4/1
  Constant/1 -> Subtract3/1
  Constant1/1 -> Subtract4/1
  Robot_Y/1 -> Subtract7/2, Subtract1/2, Subtract3/2, Subtract5/2
  Robot_X/1 -> Subtract8/2, Subtract6/2, Subtract2/2, Subtract4/2
  Field_X/1 -> Subtract8/1, Subtract2/1
  Constant2/1 -> Subtract1/1
  Field_Y/1 -> Subtract7/1, Subtract5/1
  Constant3/1 -> Subtract6/1

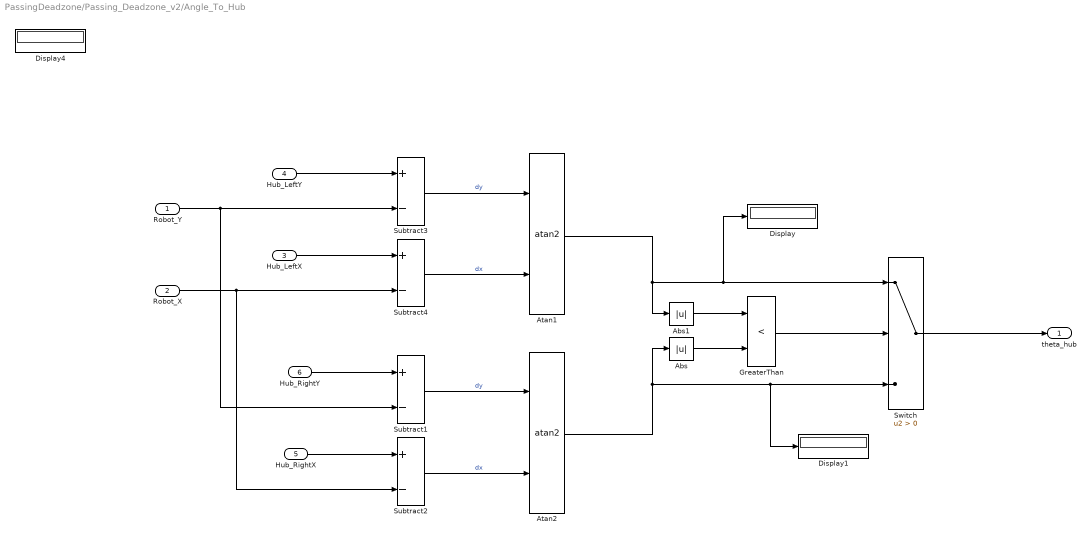
== system PassingDeadzone/Passing_Deadzone_v2/Angle_To_Hub ==
  Robot_Y : Inport
  Robot_X : Inport  Port=2
  Hub_LeftX : Inport  Port=3
  Hub_LeftY : Inport  Port=4
  Hub_RightX : Inport  Port=5
  Hub_RightY : Inport  Port=6
  Abs : Abs  SaturateOnIntegerOverflow=off
  Abs1 : Abs  SaturateOnIntegerOverflow=off
  Atan1 : Trigonometry  Operator=atan2
  Atan2 : Trigonometry  Operator=atan2
  Display : Display
  Display1 : Display
  Display4 : Display
  GreaterThan : RelationalOperator  Operator=<  OutDataTypeStr=boolean  RndMeth=Simplest  InputSameDT=off
  Subtract{1..4} (4 alike) : Sum  Inputs=+-
  Switch : Switch  Criteria=u2 > Threshold  SaturateOnIntegerOverflow=off  InputSameDT=off
  theta_hub : Outport
  wires:
  Subtract4/1 -> Atan1/2  "dx"
  Subtract3/1 -> Atan1/1  "dy"
  Robot_Y/1 -> Subtract3/2, Subtract1/2
  Robot_X/1 -> Subtract4/2, Subtract2/2
  Hub_LeftY/1 -> Subtract3/1
  Hub_LeftX/1 -> Subtract4/1
  Subtract1/1 -> Atan2/1  "dy"
  Subtract2/1 -> Atan2/2  "dx"
  Hub_RightX/1 -> Subtract2/1
  Hub_RightY/1 -> Subtract1/1
  Atan2/1 -> Display1/1, Switch/3, Abs/1
  Atan1/1 -> Display/1, Switch/1, Abs1/1
  GreaterThan/1 -> Switch/2
  Switch/1 -> theta_hub/1
  Abs1/1 -> GreaterThan/1
  Abs/1 -> GreaterThan/2

== system PassingDeadzone/Passing_Deadzone_v2/Choose_Corner ==
  theta_cor1 : Inport
  theta_cor2 : Inport  Port=2
  theta_cor3 : Inport  Port=3
  theta_cor4 : Inport  Port=4
  Target_X : Inport  Port=5
  Target_Y : Inport  Port=6
  If : If  IfExpression=u1 > Field_Hub_Y
  If Action Subsystem : Subsystem  TreatAsAtomicUnit=on
  If Action Subsystem1 : Subsystem  TreatAsAtomicUnit=on
  Merge : Merge
  theta_corner : Outport
  wires:
  If/1 -> If Action Subsystem/Action
  Target_Y/1 -> If/1
  If/2 -> If Action Subsystem1/Action
  theta_cor1/1 -> If Action Subsystem1/1(theta_cor1)
  If Action Subsystem/1(theta_corner) -> Merge/1
  If Action Subsystem1/1(theta_corner) -> Merge/2
  Merge/1 -> theta_corner/1
  Target_X/1 -> If Action Subsystem1/3(Target_X), If Action Subsystem/3(Target_X)
  theta_cor2/1 -> If Action Subsystem1/2(theta_cor2)
  theta_cor3/1 -> If Action Subsystem/1(theta_cor3)
  theta_cor4/1 -> If Action Subsystem/2(theta_cor4)

== system PassingDeadzone/Passing_Deadzone_v2/Choose_Hub ==
  Blue_Hub_LeftX : Inport
  Blue_Hub_LeftY : Inport  Port=2
  Blue_Hub_RightX : Inport  Port=3
  Blue_Hub_RightY : Inport  Port=4
  Red_Hub_LeftX : Inport  Port=5
  Red_Hub_LeftY : Inport  Port=6
  Red_Hub_RightX : Inport  Port=7
  Red_Hub_RightY : Inport  Port=8
  IsBlueAlliance : Inport  Port=9
  Switch{,1..3} (4 alike) : Switch  Criteria=u2 > Threshold  SaturateOnIntegerOverflow=off  InputSameDT=off
  Hub_LeftX : Outport
  Hub_LeftY : Outport  Port=2
  Hub_RightX : Outport  Port=3
  Hub_RightY : Outport  Port=4
  wires:
  IsBlueAlliance/1 -> Switch/2, Switch1/2, Switch2/2, Switch3/2
  Switch/1 -> Hub_LeftX/1
  Switch1/1 -> Hub_LeftY/1
  Switch2/1 -> Hub_RightY/1
  Switch3/1 -> Hub_RightX/1
  Blue_Hub_LeftX/1 -> Switch/1
  Red_Hub_LeftY/1 -> Switch1/3
  Blue_Hub_LeftY/1 -> Switch1/1
  Blue_Hub_RightX/1 -> Switch2/1
  Red_Hub_RightX/1 -> Switch2/3
  Red_Hub_RightY/1 -> Switch3/3
  Blue_Hub_RightY/1 -> Switch3/1
  Red_Hub_LeftX/1 -> Switch/3

== system PassingDeadzone/Passing_Deadzone_v2/Subsystem ==
  Target_Y : Inport
  Robot_Y : Inport  Port=2
  Target_X : Inport  Port=3
  Robot_X : Inport  Port=4
  Desired_Shot_Distance : Inport  Port=5
  Add : Sum  Inputs=+++
  Atan2 : Trigonometry  Operator=atan2
  Constant : Constant  Value=Rebuilt_Des_Gyro_Shoot_Offset
  Degrees to Radians : simulink_extras/Transformations/Degrees to Radians
  Divide : Product  Inputs=*/
  Max : MinMax  Function=max  Inputs=2
  Shooter Assembly Offset in Robot : Constant  Value=-2.94*0.0254
  Shooter Assembly Offset in Robot1 : Constant  Value=0.001
  Subtract1 : Sum  Inputs=+-
  Subtract2 : Sum  Inputs=+-
  Tanh1 : Trigonometry  Operator=atan
  PassAngle : Outport
  wires:
  Target_X/1 -> Subtract2/1
  Subtract2/1 -> Atan2/2  "dx"
  Subtract1/1 -> Atan2/1  "dy"
  Target_Y/1 -> Subtract1/1
  Robot_X/1 -> Subtract2/2
  Robot_Y/1 -> Subtract1/2
  Max/1 -> Divide/2
  Shooter Assembly Offset in Robot/1 -> Divide/1
  Shooter Assembly Offset in Robot1/1 -> Max/2
  Divide/1 -> Tanh1/1
  Desired_Shot_Distance/1 -> Max/1
  Tanh1/1 -> Add/2
  Constant/1 -> Degrees to Radians/1
  Add/1 -> PassAngle/1
  Atan2/1 -> Add/1
  Degrees to Radians/1 -> Add/3

== system PassingDeadzone/Passing_Deadzone_v2/Subsystem1 ==
  theta_corner : Inport
  theta_hub : Inport  Port=2
  IsBlueAlliance : Inport  Port=3
  Gyro_Angle_Field : Inport  Port=4
  AND : Logic  AllPortsSameDT=off  OutDataTypeStr=boolean
  AND1 : Logic  AllPortsSameDT=off  OutDataTypeStr=boolean
  GreaterThan : RelationalOperator  Operator=<  OutDataTypeStr=boolean  RndMeth=Simplest  InputSameDT=off
  GreaterThan1 : RelationalOperator  Operator=>  OutDataTypeStr=boolean  RndMeth=Simplest  InputSameDT=off
  GreaterThan2 : RelationalOperator  Operator=<  OutDataTypeStr=boolean  RndMeth=Simplest  InputSameDT=off
  GreaterThan3 : RelationalOperator  Operator=>  OutDataTypeStr=boolean  RndMeth=Simplest  InputSameDT=off
  GreaterThan4 : RelationalOperator  Operator=<  OutDataTypeStr=boolean  RndMeth=Simplest  InputSameDT=off
  Logical Operator : Logic  Operator=NXOR  AllPortsSameDT=off  OutDataTypeStr=boolean
  Switch : Switch  Criteria=u2 > Threshold  SaturateOnIntegerOverflow=off  InputSameDT=off
  Can_Bot_Pass : Outport
  wires:
  theta_corner/1 -> GreaterThan1/2, GreaterThan4/2, GreaterThan/1
  theta_hub/1 -> GreaterThan2/2, GreaterThan3/2, GreaterThan/2
  Gyro_Angle_Field/1 -> GreaterThan4/1, GreaterThan3/1, GreaterThan2/1, GreaterThan1/1
  GreaterThan1/1 -> AND/1
  GreaterThan2/1 -> AND/2
  GreaterThan3/1 -> AND1/1
  GreaterThan4/1 -> AND1/2
  AND/1 -> Switch/1
  AND1/1 -> Switch/3
  GreaterThan/1 -> Switch/2
  IsBlueAlliance/1 -> Logical Operator/1
  Switch/1 -> Logical Operator/2
  Logical Operator/1 -> Can_Bot_Pass/1

== system PassingDeadzone/Passing_Deadzone/Choose_Corner/If Action Subsystem ==
  theta_cor3 : Inport
  theta_cor4 : Inport  Port=2
  Target_X : Inport  Port=3
  Action Port : ActionPort  ActionPortLabel=if(u1 > Field_Hub_Y)
  Switch : Switch  Criteria=u2 > Threshold  Threshold=Field_Length_Half  SaturateOnIntegerOverflow=off  InputSameDT=off
  theta_corner : Outport
  wires:
  Target_X/1 -> Switch/2
  theta_cor4/1 -> Switch/1
  theta_cor3/1 -> Switch/3
  Switch/1 -> theta_corner/1

== system PassingDeadzone/Passing_Deadzone/Choose_Corner/If Action Subsystem1 ==
  theta_cor1 : Inport
  theta_cor2 : Inport  Port=2
  Target_X : Inport  Port=3
  Action Port : ActionPort  ActionPortLabel=else
  Switch : Switch  Criteria=u2 > Threshold  Threshold=Field_Length_Half  SaturateOnIntegerOverflow=off  InputSameDT=off
  theta_corner : Outport
  wires:
  Target_X/1 -> Switch/2
  theta_cor2/1 -> Switch/1
  theta_cor1/1 -> Switch/3
  Switch/1 -> theta_corner/1

== system PassingDeadzone/Passing_Deadzone1/Choose_Corner/If Action Subsystem ==
  theta_cor3 : Inport
  theta_cor4 : Inport  Port=2
  Target_X : Inport  Port=3
  Action Port : ActionPort  ActionPortLabel=if(u1 > Field_Hub_Y)
  Switch : Switch  Criteria=u2 > Threshold  Threshold=Field_Length_Half  SaturateOnIntegerOverflow=off  InputSameDT=off
  theta_corner : Outport
  wires:
  Target_X/1 -> Switch/2
  theta_cor4/1 -> Switch/1
  theta_cor3/1 -> Switch/3
  Switch/1 -> theta_corner/1

== system PassingDeadzone/Passing_Deadzone1/Choose_Corner/If Action Subsystem1 ==
  theta_cor1 : Inport
  theta_cor2 : Inport  Port=2
  Target_X : Inport  Port=3
  Action Port : ActionPort  ActionPortLabel=else
  Switch : Switch  Criteria=u2 > Threshold  Threshold=Field_Length_Half  SaturateOnIntegerOverflow=off  InputSameDT=off
  theta_corner : Outport
  wires:
  Target_X/1 -> Switch/2
  theta_cor2/1 -> Switch/1
  theta_cor1/1 -> Switch/3
  Switch/1 -> theta_corner/1

== system PassingDeadzone/Passing_Deadzone_v2/Choose_Corner/If Action Subsystem ==
  theta_cor3 : Inport
  theta_cor4 : Inport  Port=2
  Target_X : Inport  Port=3
  Action Port : ActionPort  ActionPortLabel=if(u1 > Field_Hub_Y)
  Switch : Switch  Criteria=u2 > Threshold  Threshold=Field_Length_Half  SaturateOnIntegerOverflow=off  InputSameDT=off
  theta_corner : Outport
  wires:
  Target_X/1 -> Switch/2
  theta_cor4/1 -> Switch/1
  theta_cor3/1 -> Switch/3
  Switch/1 -> theta_corner/1

== system PassingDeadzone/Passing_Deadzone_v2/Choose_Corner/If Action Subsystem1 ==
  theta_cor1 : Inport
  theta_cor2 : Inport  Port=2
  Target_X : Inport  Port=3
  Action Port : ActionPort  ActionPortLabel=else
  Switch : Switch  Criteria=u2 > Threshold  Threshold=Field_Length_Half  SaturateOnIntegerOverflow=off  InputSameDT=off
  theta_corner : Outport
  wires:
  Target_X/1 -> Switch/2
  theta_cor2/1 -> Switch/1
  theta_cor1/1 -> Switch/3
  Switch/1 -> theta_corner/1
